simulink model "sm_car"  (R2025a)
settings: Solver=ode23t  StartTime=0.0  StopTime=400  MaxStep=0.4  RelTol=1e-3  AbsTol=1e-3  EnableMultiTasking=on
PreLoadFcn:
  | % Due to usability issue in Repeating Sequence block
  | warning('off','Simulink:Masking:Invalid');
  | 
  | % Eliminate unnecessary warnings in inactive variants
  | % Warnings generated only if you click through inactive variant
  | warning('off','MATLAB:nonExistentField');
  | warning('off','Simulink:Parameters:BlkParamUndefined');
PostLoadFcn:
  | set_param([bdroot '/Vehicle'],'popup_trailer','Off')
  | warning('off','sm:sli:setup:compile:LocalSolverNotSupported')
  | %sm_car_config_maneuver(bdroot,'WOT Braking');
  | sm_car_config_vehicle(bdroot,'false');
  | sm_car_config_logging(bdroot);
InitFcn:
  | sm_car_config_camera;
  | Vehicle = sm_car_vehcfg_checkConfig(Vehicle);
  | sm_car_check_tire_model(bdroot);
StartFcn:
  | tic;
StopFcn:
  | Elapsed_Sim_Time = toc;
  | % disp(['Elapsed Sim Time = ' num2str(Elapsed_Sim_Time)]);
undefined symbols (not defined in the file): Axle1D, AxleIn, Camera, Control, Driver, Free, Init, Maneuver, Pedal, RaceFix, RaceSpin, Scene, ShaftL1, ShaftL2, ShaftR1, ShaftR2, Soft, Stiff, Visual, X, xy_data_car_side, Y, Z
libraries: sm_lib x1546, nesl_utility x528, fl_lib x480, SimscapeFluids_lib x61, sdl_lib x49, simulink x29, ee_lib x7, simulink_extras x6, Linkage_Systems x4, Tire_1x2x x4, AntiRollBar_Systems x2, Linkage_Decoupled x2
(part 55 of 79)

== system sm_car/Vehicle/Vehicle/Chassis/SuspA1/Linkage Decoupled/Steer/Wheel Driven Rack 1UJoint/Steer Mount ==
  note: Two additional degrees of freedom have been added
      | to ensure steering column assembles within tolerances.
  Cylindrical Joint : sm_lib/Joints/Cylindrical Joint  JointMode=Normal  CompositeWrenchDir=FollowerOnBase  CompositeWrenchFrame=BaseFrame  SenseConstraintForce=off  SenseConstraintTorque=off  SenseTotalForce=off  SenseTotalTorque=off  RzPositionTargetSpecify=off  RzPositionTargetPriority=High  RzPositionTargetValue=0  RzPositionTargetValueUnits=deg  RzVelocityTargetSpecify=off  RzVelocityTargetPriority=High  RzVelocityTargetValue=0  RzVelocityTargetValueUnits=deg/s  RzEquilibriumPosition=0  RzEquilibriumPositionUnits=deg  RzSpringStiffness=0  RzSpringStiffnessUnits=N*m/deg  RzDampingCoefficient=0  RzDampingCoefficientUnits=N*m/(deg/s)  RzLowerLimitSpecify=off  RzLowerLimitBound=-90  RzLowerLimitBoundUnits=deg  RzLowerLimitStiffness=1e4  RzLowerLimitStiffnessUnits=N*m/deg  RzLowerLimitDamping=10  RzLowerLimitDampingUnits=N*m/(deg/s)  RzLowerLimitTransitionRegionWidth=0.1  RzLowerLimitTransitionRegionWidthUnits=deg  RzUpperLimitSpecify=off  RzUpperLimitBound=90  RzUpperLimitBoundUnits=deg  RzUpperLimitStiffness=1e4  RzUpperLimitStiffnessUnits=N*m/deg  RzUpperLimitDamping=10  RzUpperLimitDampingUnits=N*m/(deg/s)  RzUpperLimitTransitionRegionWidth=0.1  RzUpperLimitTransitionRegionWidthUnits=deg  RzTorqueActuationMode=ComputedTorque  RzMotionActuationMode=InputMotion  RzSensePosition=on  RzSenseVelocity=off  RzSenseAcceleration=off  RzSenseTorqueForce=off  RzSenseLowerLimitTorqueForce=off  RzSenseUpperLimitTorqueForce=off  PzPositionTargetSpecify=off  PzPositionTargetPriority=High  PzPositionTargetValue=0  PzPositionTargetValueUnits=m  PzVelocityTargetSpecify=off  PzVelocityTargetPriority=High  PzVelocityTargetValue=0  PzVelocityTargetValueUnits=m/s  PzEquilibriumPosition=0  PzEquilibriumPositionUnits=m  PzSpringStiffness=0  PzSpringStiffnessUnits=N/m  PzDampingCoefficient=0  PzDampingCoefficientUnits=N/(m/s)  PzLowerLimitSpecify=off  PzLowerLimitBound=-1  PzLowerLimitBoundUnits=m  PzLowerLimitStiffness=1e6  PzLowerLimitStiffnessUnits=N/m  PzLowerLimitDamping=1e3  PzLowerLimitDampingUnits=N/(m/s)  PzLowerLimitTransitionRegionWidth=1e-4  PzLowerLimitTransitionRegionWidthUnits=m  PzUpperLimitSpecify=off  PzUpperLimitBound=1  PzUpperLimitBoundUnits=m  PzUpperLimitStiffness=1e6  PzUpperLimitStiffnessUnits=N/m  PzUpperLimitDamping=1e3  PzUpperLimitDampingUnits=N/(m/s)  PzUpperLimitTransitionRegionWidth=1e-4  PzUpperLimitTransitionRegionWidthUnits=m  PzTorqueActuationMode=NoTorque  PzMotionActuationMode=ComputedMotion  PzSensePosition=off  PzSenseVelocity=off  PzSenseAcceleration=off  PzSenseTorqueForce=off  PzSenseLowerLimitTorqueForce=off  PzSenseUpperLimitTorqueForce=off
  Revolute Joint : sm_lib/Joints/Revolute Joint  JointMode=Normal  CompositeWrenchDir=FollowerOnBase  CompositeWrenchFrame=BaseFrame  SenseConstraintForce=off  SenseConstraintTorque=off  SenseTotalForce=off  SenseTotalTorque=off  PositionTargetSpecify=off  PositionTargetPriority=High  PositionTargetValue=0  PositionTargetValueUnits=deg  VelocityTargetSpecify=off  VelocityTargetPriority=High  VelocityTargetValue=0  VelocityTargetValueUnits=deg/s  EquilibriumPosition=0  EquilibriumPositionUnits=deg  SpringStiffness=0  SpringStiffnessUnits=N*m/deg  DampingCoefficient=0  DampingCoefficientUnits=N*m/(deg/s)  LowerLimitSpecify=off  LowerLimitBound=-90  LowerLimitBoundUnits=deg  LowerLimitStiffness=1e4  LowerLimitStiffnessUnits=N*m/deg  LowerLimitDamping=10  LowerLimitDampingUnits=N*m/(deg/s)  LowerLimitTransitionRegionWidth=0.1  LowerLimitTransitionRegionWidthUnits=deg  UpperLimitSpecify=off  UpperLimitBound=90  UpperLimitBoundUnits=deg  UpperLimitStiffness=1e4  UpperLimitStiffnessUnits=N*m/deg  UpperLimitDamping=10  UpperLimitDampingUnits=N*m/(deg/s)  UpperLimitTransitionRegionWidth=0.1  UpperLimitTransitionRegionWidthUnits=deg  TorqueActuationMode=NoTorque  MotionActuationMode=ComputedMotion  SensePosition=off  SenseVelocity=off  SenseAcceleration=off  SenseTorqueForce=off  SenseLowerLimitTorqueForce=off  SenseUpperLimitTorqueForce=off
  Transform DOF wy B : sm_lib/Frames and Transforms/Rigid Transform  RotationMethod=StandardAxis  FollAlignAxisA=+X  BaseAlignAxisA=+Y  FollAlignAxisB=+Y  BaseAlignAxisB=+Z  RotationStandardAxis=+X  RotationAngle=-90  RotationAngleUnits=deg  RotationArbitraryAxis=[0 0 1]  RotationSequenceAxes=FollowerAxes  RotationSequence=XYX  RotationSequenceAngles=[0 0 0]  RotationSequenceAnglesUnits=deg  RotationMatrix=[1 0 0; 0 1 0; 0 0 1]  Quaternion=[1 0 0 0]  TranslationMethod=None  TranslationCartesianOffset=[0 0 0]  TranslationCartesianOffsetUnits=m  TranslationStandardAxis=+Z  TranslationStandardOffset=0  TranslationStandardOffsetUnits=m  TranslationROffset=0  TranslationROffsetUnits=m  TranslationThetaOffset=0  TranslationThetaOffsetUnits=deg  TranslationZOffset=0  TranslationZOffsetUnits=m
  Transform DOF wy F : sm_lib/Frames and Transforms/Rigid Transform  RotationMethod=StandardAxis  FollAlignAxisA=+X  BaseAlignAxisA=+Y  FollAlignAxisB=+Y  BaseAlignAxisB=+Z  RotationStandardAxis=+X  RotationAngle=-90  RotationAngleUnits=deg  RotationArbitraryAxis=[0 0 1]  RotationSequenceAxes=FollowerAxes  RotationSequence=XYX  RotationSequenceAngles=[0 0 0]  RotationSequenceAnglesUnits=deg  RotationMatrix=[1 0 0; 0 1 0; 0 0 1]  Quaternion=[1 0 0 0]  TranslationMethod=None  TranslationCartesianOffset=[0 0 0]  TranslationCartesianOffsetUnits=m  TranslationStandardAxis=+Z  TranslationStandardOffset=0  TranslationStandardOffsetUnits=m  TranslationROffset=0  TranslationROffsetUnits=m  TranslationThetaOffset=0  TranslationThetaOffsetUnits=deg  TranslationZOffset=0  TranslationZOffsetUnits=m
  F : PMIOPort  Side=Right
  B : PMIOPort  Port=2  Side=Left
  a : PMIOPort  Port=3  Side=Right
  q : PMIOPort  Port=4  Side=Left
  connections:
  a/RConn1 -- Cylindrical Joint/RConn2
  q/RConn1 -- Cylindrical Joint/LConn2
  Transform DOF wy B/LConn1 -- B/RConn1
  Cylindrical Joint/RConn1 -- F/RConn1
  Cylindrical Joint/LConn1 -- Transform DOF wy F/LConn1
  Revolute Joint/LConn1 -- Transform DOF wy B/RConn1
  Transform DOF wy F/RConn1 -- Revolute Joint/RConn1

== system sm_car/Vehicle/Vehicle/Chassis/SuspA1/Linkage Decoupled/Steer/Wheel Driven Rack 1UJoint/Wheel ==
  FSAE : Subsystem  VariantControl=FSAE
  Sedan : Subsystem  VariantControl=Sedan  mask{clr_wheel=Visual.SteeringWheel.clr, opc_wheel=1}
      mask prompts: clr_wheel "Color [RGB]"; opc_wheel "Opacity (0-1)"
  SteerAxis : PMIOPort  Side=Left
  HandR : PMIOPort  Port=2  Side=Right
  HandL : PMIOPort  Port=3  Side=Right

== system sm_car/Vehicle/Vehicle/Chassis/SuspA2/Linkage/Steer/None/Body Sensor ==
  note: Calculation not yet implemented
  Constant : Constant  Value=0
  Constant1 : Constant  Value=0
  PS-Simulink Converter1 : nesl_utility/PS-Simulink Converter  PhysicalDomain=network_engine_domain  SubClassName=ps_output  LeftPortType=input  RightPortType=output  PseudoPeriodic=off  Frequencies=[]  VectorFormat=1-D array  Unit=m  AffineConversion=off
  PS-Simulink Converter11 : nesl_utility/PS-Simulink Converter  PhysicalDomain=network_engine_domain  SubClassName=ps_output  LeftPortType=input  RightPortType=output  PseudoPeriodic=off  Frequencies=[]  VectorFormat=1-D array  Unit=1  AffineConversion=off
  PS-Simulink Converter2 : nesl_utility/PS-Simulink Converter  PhysicalDomain=network_engine_domain  SubClassName=ps_output  LeftPortType=input  RightPortType=output  PseudoPeriodic=off  Frequencies=[]  VectorFormat=1-D array  Unit=m  AffineConversion=off
  PS-Simulink Converter3 : nesl_utility/PS-Simulink Converter  PhysicalDomain=network_engine_domain  SubClassName=ps_output  LeftPortType=input  RightPortType=output  PseudoPeriodic=off  Frequencies=[]  VectorFormat=1-D array  Unit=m  AffineConversion=off
  PS-Simulink Converter4 : nesl_utility/PS-Simulink Converter  PhysicalDomain=network_engine_domain  SubClassName=ps_output  LeftPortType=input  RightPortType=output  PseudoPeriodic=off  Frequencies=[]  VectorFormat=1-D array  Unit=m/s  AffineConversion=off
  PS-Simulink Converter5 : nesl_utility/PS-Simulink Converter  PhysicalDomain=network_engine_domain  SubClassName=ps_output  LeftPortType=input  RightPortType=output  PseudoPeriodic=off  Frequencies=[]  VectorFormat=1-D array  Unit=m/s  AffineConversion=off
  PS-Simulink Converter6 : nesl_utility/PS-Simulink Converter  PhysicalDomain=network_engine_domain  SubClassName=ps_output  LeftPortType=input  RightPortType=output  PseudoPeriodic=off  Frequencies=[]  VectorFormat=1-D array  Unit=m/s  AffineConversion=off
  PS-Simulink Converter7 : nesl_utility/PS-Simulink Converter  PhysicalDomain=network_engine_domain  SubClassName=ps_output  LeftPortType=input  RightPortType=output  PseudoPeriodic=off  Frequencies=[]  VectorFormat=1-D array  Unit=m/s^2  AffineConversion=off
  PS-Simulink Converter8 : nesl_utility/PS-Simulink Converter  PhysicalDomain=network_engine_domain  SubClassName=ps_output  LeftPortType=input  RightPortType=output  PseudoPeriodic=off  Frequencies=[]  VectorFormat=1-D array  Unit=m/s^2  AffineConversion=off
  PS-Simulink Converter9 : nesl_utility/PS-Simulink Converter  PhysicalDomain=network_engine_domain  SubClassName=ps_output  LeftPortType=input  RightPortType=output  PseudoPeriodic=off  Frequencies=[]  VectorFormat=1-D array  Unit=m/s^2  AffineConversion=off
  Roll Pitch : Subsystem
  Signal Specification : SignalSpecification  Unit=rad
  Signal Specification1 : SignalSpecification  Unit=rad
  Signal Specification2 : SignalSpecification  Unit=rad
  Signal Specification3 : SignalSpecification  Unit=rad/s
  Signal Specification4 : SignalSpecification  Unit=rad/s
  Signal Specification5 : SignalSpecification  Unit=rad/s
  Transform Sensor Offset : sm_lib/Frames and Transforms/Rigid Transform  RotationMethod=None  FollAlignAxisA=+X  BaseAlignAxisA=+Y  FollAlignAxisB=+Y  BaseAlignAxisB=+Z  RotationStandardAxis=+Z  RotationAngle=0.0  RotationAngleUnits=deg  RotationArbitraryAxis=[0 0 1]  RotationSequenceAxes=FollowerAxes  RotationSequence=XYX  RotationSequenceAngles=[0 0 0]  RotationSequenceAnglesUnits=deg  RotationMatrix=[1 0 0; 0 1 0; 0 0 1]  Quaternion=[1 0 0 0]  TranslationMethod=Cartesian  TranslationCartesianOffset=offset_body_sensor  TranslationCartesianOffsetUnits=m  TranslationStandardAxis=+Z  TranslationStandardOffset=0  TranslationStandardOffsetUnits=m  TranslationROffset=0  TranslationROffsetUnits=m  TranslationThetaOffset=0  TranslationThetaOffsetUnits=deg  TranslationZOffset=0  TranslationZOffsetUnits=m
  Transform Sensor Body : sm_lib/Frames and Transforms/Transform Sensor  MeasurementFrame=NonRotatingFollower  RotationSequence=XYX  SenseAngle=off  SenseAxis=off  SenseQ=off  SenseR=on  SenseRotationSequence=off  SenseOmegaX=off  SenseOmegaY=off  SenseOmegaZ=off  SenseOmega=off  SenseQDot=off  SenseRDot=off  SenseRotationSequenceDot=off  SenseAlphaX=off  SenseAlphaY=off  SenseAlphaZ=off  SenseAlpha=off  SenseQDDot=off  SenseRDDot=off  SenseX=on  SenseY=on  SenseZ=on  SenseXYZ=off  SenseRad=off  SenseAzim=off  SenseDist=off  SenseInc=off  SenseXDot=on  SenseYDot=on  SenseZDot=on  SenseXYZDot=off  SenseRadDot=off  SenseAzimDot=off  SenseDistDot=off  SenseIncDot=off  SenseXDDot=on  SenseYDDot=on  SenseZDDot=on  SenseXYZDDot=off  SenseRadDDot=off  SenseAzimDDot=off  SenseDistDDot=off  SenseIncDDot=off
  World Frame : sm_lib/Frames and Transforms/World Frame
  B : PMIOPort  Side=Left
  Bus Element Out : Outport  VectorParamsAs1DForOutWhenUnconnected=off  PortName=Body  Element=x
  Bus Element Out1 : Outport  VectorParamsAs1DForOutWhenUnconnected=off  PortName=Body  Element=y
  Bus Element Out2 : Outport  VectorParamsAs1DForOutWhenUnconnected=off  PortName=Body  Element=z
  Bus Element Out3 : Outport  VectorParamsAs1DForOutWhenUnconnected=off  PortName=Body  Element=vx
  Bus Element Out4 : Outport  VectorParamsAs1DForOutWhenUnconnected=off  PortName=Body  Element=vy
  Bus Element Out5 : Outport  VectorParamsAs1DForOutWhenUnconnected=off  PortName=Body  Element=vz
  Bus Element Out6 : Outport  VectorParamsAs1DForOutWhenUnconnected=off  PortName=Body  Element=gx
  Bus Element Out7 : Outport  VectorParamsAs1DForOutWhenUnconnected=off  PortName=Body  Element=gy
  Bus Element Out8 : Outport  VectorParamsAs1DForOutWhenUnconnected=off  PortName=Body  Element=gz
  Bus Element Out9 : Outport  VectorParamsAs1DForOutWhenUnconnected=off  PortName=Body  Element=nRoll
  Bus Element Out10 : Outport  VectorParamsAs1DForOutWhenUnconnected=off  PortName=Body  Element=nPitch
  Bus Element Out11 : Outport  VectorParamsAs1DForOutWhenUnconnected=off  PortName=Body  Element=nYaw
  Bus Element Out12 : Outport  VectorParamsAs1DForOutWhenUnconnected=off  PortName=Body  Element=aRoll
  Bus Element Out13 : Outport  VectorParamsAs1DForOutWhenUnconnected=off  PortName=Body  Element=aPitch
  Bus Element Out14 : Outport  VectorParamsAs1DForOutWhenUnconnected=off  PortName=Body  Element=aYaw
  wires:
  PS-Simulink Converter9/1 -> Bus Element Out8/1
  PS-Simulink Converter11/1 -> Roll Pitch/1(R)
  PS-Simulink Converter6/1 -> Bus Element Out5/1
  PS-Simulink Converter7/1 -> Bus Element Out6/1
  PS-Simulink Converter2/1 -> Bus Element Out1/1
  PS-Simulink Converter8/1 -> Bus Element Out7/1
  PS-Simulink Converter5/1 -> Bus Element Out4/1
  PS-Simulink Converter3/1 -> Bus Element Out2/1
  PS-Simulink Converter1/1 -> Bus Element Out/1
  PS-Simulink Converter4/1 -> Bus Element Out3/1
  Signal Specification/1 -> Bus Element Out12/1
  Signal Specification1/1 -> Bus Element Out13/1
  Signal Specification2/1 -> Bus Element Out14/1
  Signal Specification3/1 -> Bus Element Out9/1
  Signal Specification4/1 -> Bus Element Out10/1
  Signal Specification5/1 -> Bus Element Out11/1
  Constant/1 -> Signal Specification2/1
  Constant1/1 -> Signal Specification5/1
  Roll Pitch/3(nRoll) -> Signal Specification3/1
  Roll Pitch/4(nPitch) -> Signal Specification4/1
  Roll Pitch/2(aPitch) -> Signal Specification1/1
  Roll Pitch/1(aRoll) -> Signal Specification/1
  connections:
  Transform Sensor Body/RConn5 -- PS-Simulink Converter3/LConn1
  Transform Sensor Body/RConn4 -- PS-Simulink Converter2/LConn1
  Transform Sensor Body/RConn11 -- PS-Simulink Converter9/LConn1
  Transform Sensor Body/RConn2 -- PS-Simulink Converter11/LConn1
  Transform Sensor Body/RConn7 -- PS-Simulink Converter5/LConn1
  Transform Sensor Body/RConn3 -- PS-Simulink Converter1/LConn1
  Transform Sensor Body/LConn1 -- World Frame/RConn1
  Transform Sensor Offset/LConn1 -- B/RConn1
  Transform Sensor Body/RConn10 -- PS-Simulink Converter8/LConn1
  Transform Sensor Body/RConn9 -- PS-Simulink Converter7/LConn1
  Transform Sensor Body/RConn8 -- PS-Simulink Converter6/LConn1
  Transform Sensor Body/RConn6 -- PS-Simulink Converter4/LConn1
  Transform Sensor Body/RConn1 -- Transform Sensor Offset/RConn1

== system sm_car/Vehicle/Vehicle/Powertrain/Power/Electric L1 R1 L2 R2/Thermal/Liquid Loop1/Pump Control ==
  T : Inport
  Memory : Memory
  Pump Time Constant : TransferFcn  Denominator=[0.1 1]
  Relay : Relay  OnSwitchValue=313  OffSwitchValue=293  ZeroCross=off
  M : Outport  VectorParamsAs1DForOutWhenUnconnected=off
  wires:
  Pump Time Constant/1 -> M/1
  Memory/1 -> Relay/1
  T/1 -> Memory/1
  Relay/1 -> Pump Time Constant/1  "Pump_flw"

== system sm_car/Vehicle/Vehicle/Powertrain/Power/Electric L1 R1 L2 R2/Thermal/Liquid Loop1/Sensing TBattery ==
  PS-Simulink Converter4 : nesl_utility/PS-Simulink Converter  PhysicalDomain=network_engine_domain  SubClassName=ps_output  LeftPortType=input  RightPortType=output  PseudoPeriodic=off  Frequencies=[]  VectorFormat=1-D array  Unit=K  AffineConversion=on
  Temperature Sensor : fl_lib/Thermal/Thermal Sensors/Temperature Sensor  temperature_measure=foundation.enum.MeasurementReference.difference
  Thermal Reference : fl_lib/Thermal/Thermal Elements/Thermal Reference
  A : PMIOPort  Side=Left
  T : Outport  VectorParamsAs1DForOutWhenUnconnected=off
  wires:
  PS-Simulink Converter4/1 -> T/1  "Temperature"
  connections:
  Temperature Sensor/LConn1 -- A/RConn1
  Thermal Reference/LConn1 -- Temperature Sensor/RConn1
  Temperature Sensor/RConn2 -- PS-Simulink Converter4/LConn1

== system sm_car/Vehicle/Vehicle/Powertrain/Power/Electric L1 R1 L2 R2/Thermal/Liquid Loop1/Sensing TConverter ==
  PS-Simulink Converter4 : nesl_utility/PS-Simulink Converter  PhysicalDomain=network_engine_domain  SubClassName=ps_output  LeftPortType=input  RightPortType=output  PseudoPeriodic=off  Frequencies=[]  VectorFormat=1-D array  Unit=K  AffineConversion=on
  Temperature Sensor : fl_lib/Thermal/Thermal Sensors/Temperature Sensor  temperature_measure=foundation.enum.MeasurementReference.difference
  Thermal Reference : fl_lib/Thermal/Thermal Elements/Thermal Reference
  A : PMIOPort  Side=Left
  T : Outport  VectorParamsAs1DForOutWhenUnconnected=off
  wires:
  PS-Simulink Converter4/1 -> T/1  "Temperature"
  connections:
  Temperature Sensor/RConn2 -- PS-Simulink Converter4/LConn1
  Thermal Reference/LConn1 -- Temperature Sensor/RConn1
  Temperature Sensor/LConn1 -- A/RConn1

== system sm_car/Vehicle/Vehicle/Powertrain/Power/Electric L1 R1 L2 R2/Thermal/Liquid Loop1/Sensing TMotorR1 ==
  PS-Simulink Converter4 : nesl_utility/PS-Simulink Converter  PhysicalDomain=network_engine_domain  SubClassName=ps_output  LeftPortType=input  RightPortType=output  PseudoPeriodic=off  Frequencies=[]  VectorFormat=1-D array  Unit=K  AffineConversion=on
  Temperature Sensor : fl_lib/Thermal/Thermal Sensors/Temperature Sensor  temperature_measure=foundation.enum.MeasurementReference.difference
  Thermal Reference : fl_lib/Thermal/Thermal Elements/Thermal Reference
  A : PMIOPort  Side=Left
  T : Outport  VectorParamsAs1DForOutWhenUnconnected=off
  wires:
  PS-Simulink Converter4/1 -> T/1  "Temperature"
  connections:
  Temperature Sensor/RConn2 -- PS-Simulink Converter4/LConn1
  Thermal Reference/LConn1 -- Temperature Sensor/RConn1
  Temperature Sensor/LConn1 -- A/RConn1

== system sm_car/Vehicle/Vehicle/Powertrain/Power/Electric L1 R1 L2 R2/Thermal/Liquid Loop1/Sensing TMotorRL ==
  PS-Simulink Converter4 : nesl_utility/PS-Simulink Converter  PhysicalDomain=network_engine_domain  SubClassName=ps_output  LeftPortType=input  RightPortType=output  PseudoPeriodic=off  Frequencies=[]  VectorFormat=1-D array  Unit=K  AffineConversion=on
  Temperature Sensor : fl_lib/Thermal/Thermal Sensors/Temperature Sensor  temperature_measure=foundation.enum.MeasurementReference.difference
  Thermal Reference : fl_lib/Thermal/Thermal Elements/Thermal Reference
  A : PMIOPort  Side=Left
  T : Outport  VectorParamsAs1DForOutWhenUnconnected=off
  wires:
  PS-Simulink Converter4/1 -> T/1  "Temperature"
  connections:
  Temperature Sensor/LConn1 -- A/RConn1
  Thermal Reference/LConn1 -- Temperature Sensor/RConn1
  Temperature Sensor/RConn2 -- PS-Simulink Converter4/LConn1

== system sm_car/Vehicle/Vehicle/Powertrain/Power/Electric L1 R1 L2 R2/Thermal/Liquid Loop1/Sensing TMotorRL1 ==
  PS-Simulink Converter4 : nesl_utility/PS-Simulink Converter  PhysicalDomain=network_engine_domain  SubClassName=ps_output  LeftPortType=input  RightPortType=output  PseudoPeriodic=off  Frequencies=[]  VectorFormat=1-D array  Unit=K  AffineConversion=on
  Temperature Sensor : fl_lib/Thermal/Thermal Sensors/Temperature Sensor  temperature_measure=foundation.enum.MeasurementReference.difference
  Thermal Reference : fl_lib/Thermal/Thermal Elements/Thermal Reference
  A : PMIOPort  Side=Left
  T : Outport  VectorParamsAs1DForOutWhenUnconnected=off
  wires:
  PS-Simulink Converter4/1 -> T/1  "Temperature"
  connections:
  Temperature Sensor/RConn2 -- PS-Simulink Converter4/LConn1
  Thermal Reference/LConn1 -- Temperature Sensor/RConn1
  Temperature Sensor/LConn1 -- A/RConn1

== system sm_car/Vehicle/Vehicle/Powertrain/Power/Electric L1 R1 L2 R2/Thermal/Liquid Loop1/Sensing TMotorRR ==
  PS-Simulink Converter4 : nesl_utility/PS-Simulink Converter  PhysicalDomain=network_engine_domain  SubClassName=ps_output  LeftPortType=input  RightPortType=output  PseudoPeriodic=off  Frequencies=[]  VectorFormat=1-D array  Unit=K  AffineConversion=on
  Temperature Sensor : fl_lib/Thermal/Thermal Sensors/Temperature Sensor  temperature_measure=foundation.enum.MeasurementReference.difference
  Thermal Reference : fl_lib/Thermal/Thermal Elements/Thermal Reference
  A : PMIOPort  Side=Left
  T : Outport  VectorParamsAs1DForOutWhenUnconnected=off
  wires:
  PS-Simulink Converter4/1 -> T/1  "Temperature"
  connections:
  Temperature Sensor/LConn1 -- A/RConn1
  Thermal Reference/LConn1 -- Temperature Sensor/RConn1
  Temperature Sensor/RConn2 -- PS-Simulink Converter4/LConn1

== system sm_car/Vehicle/Vehicle/Powertrain/Power/Electric L1 R1 L2 R2/Thermal/Liquid Loop1/Tank ==
  Absolute Reference (TL) : fl_lib/Thermal Liquid/Elements/Absolute Reference (TL)
  Cap (G) : fl_lib/Gas/Elements/Cap (G)  p_specify=off  p_priority=None  p=0.101325 MPa  p_nominal_specify=off  p_nominal_value=1  p_nominal_unit=MPa  T_specify=off  T_priority=None  T=293.15 K  T_nominal_specify=off  T_nominal_value=1  T_nominal_unit=K
  Convective Heat Transfer : fl_lib/Thermal/Thermal Elements/Convective Heat Transfer  thermal_type=foundation.enum.constant_variable.constant  area=1 m^2  heat_tr_coeff=20 W/(m^2 * K)  min_heat_tr_coeff=1e-3 W/(K*m^2)  T_specify=off  T_priority=None  T=0 K  T_nominal_specify=off  T_nominal_value=1  T_nominal_unit=K  Q_specify=off  Q_priority=None  Q=0 W  Q_nominal_specify=off  Q_nominal_value=1  Q_nominal_unit=W
  Convective Heat Transfer1 : fl_lib/Thermal/Thermal Elements/Convective Heat Transfer  thermal_type=foundation.enum.constant_variable.constant  area=1 m^2  heat_tr_coeff=200 W/(m^2 * K)  min_heat_tr_coeff=1e-3 W/(K*m^2)  T_specify=off  T_priority=None  T=0 K  T_nominal_specify=off  T_nominal_value=1  T_nominal_unit=K  Q_specify=off  Q_priority=None  Q=0 W  Q_nominal_specify=off  Q_nominal_value=1  Q_nominal_unit=W
  PS Terminator : fl_lib/Physical Signals/Sinks/PS Terminator
  PS Terminator1 : fl_lib/Physical Signals/Sinks/PS Terminator
  PS Terminator2 : fl_lib/Physical Signals/Sinks/PS Terminator
  Reservoir (G) : fl_lib/Gas/Elements/Reservoir (G)  pressure_spec=1  reservoir_pressure=0.101325 MPa  reservoir_temperature=25 degC  area_A=0.001 m^2
  Sensor P T : fl_lib/Thermal Liquid/Sensors/Pressure & Temperature Sensor (TL)  reference=foundation.enum.MeasurementReference.difference  pressure=true  pressure_spec=foundation.enum.PressureMeasementSpec.Absolute  temperature=true
      settings: InternalSimscapePortConfiguration="{\"Bottom\":[{\"id\":\"T\",\"label\":\"T\",\"type\":\"output\"}],\"Left\":[{\"id\":\"A\",\"label\":\"A\",\"type\":\"foundation.thermal_liquid.thermal_liquid\"}],\"Right\":[{\"id\":\"B\",\"label\":\"B\",\"type\":\"foundation.thermal_liquid.thermal_liquid\"},{\"id\":\"P\",\"label\":\"P\",\"type\":\"output\"}],\"Top\":[]}"
  Tank : SimscapeFluids_lib/Thermal Liquid/Tanks & Accumulators/Tank (G-TL)  num_inlet=2  volume_total=0.01 m^3  volume_spec=1  tank_area=0.005 m^2  level_TLU=[0, 3, 5] m  volume_TLU=[0, 4, 6] m^3  inlet_areas_A1B1=[.001, .001] m^2  inlet_height_A2=0.1 m  inlet_area_A2=0.01 m^2  inlet_heights_A2B2=[.01, 0.01] m  inlet_areas_A2B2=[0.01^2/4*pi, 0.01^2/4*pi] m^2  inlet_heights_A2B2C2=[.1, .1, .1] m  inlet_areas_A2B2C2=[.01, .01, .01] m^2  inlet_heights_A2B2C2D2=0.1 * ones(1, 4) m  inlet_areas_A2B2C2D2=0.01 * ones(1, 4) m^2  inlet_heights_A2B2C2D2E2=0.1 * ones(1, 5) m  inlet_areas_A2B2C2D2E2=0.01 * ones(1, 5) m^2  inlet_heights_A2B2C2D2E2F2=0.1 * ones(1, 6) m  inlet_areas_A2B2C2D2E2F2=0.01 * ones(1, 6) m^2  capacity_check=0  max_liquid_capacity=0.01 m^3  g=9.81 m/s^2  level_specify=on  level_priority=High  level=0.1 m  level_nominal_specify=off  level_nominal_value=1  level_nominal_unit=m  volume_liquid_specify=off  volume_liquid_priority=None  volume_liquid=5 m^3  volume_liquid_nominal_specify=off  volume_liquid_nominal_value=1  volume_liquid_nominal_unit=m^3  mass_liquid_specify=off  mass_liquid_priority=None  mass_liquid=5e+3 kg  mass_liquid_nominal_specify=off  mass_liquid_nominal_value=1  mass_liquid_nominal_unit=kg  T_liquid_specify=on  T_liquid_priority=High  T_liquid=278 K  T_liquid_nominal_specify=off  T_liquid_nominal_value=1  T_liquid_nominal_unit=K  p_gas_specify=off  p_gas_priority=High  p_gas=0.101325 MPa  p_gas_nominal_specify=off  p_gas_nominal_value=1  p_gas_nominal_unit=MPa  T_gas_specify=on  T_gas_priority=High  T_gas=278 K  T_gas_nominal_specify=off  T_gas_nominal_value=1  T_gas_nominal_unit=K  rho_gas_specify=off  rho_gas_priority=None  rho_gas=1.2 kg/m^3  rho_gas_nominal_specify=off  rho_gas_nominal_value=1  rho_gas_nominal_unit=kg/m^3
      settings: InternalSimscapePortConfiguration="{\"Bottom\":[],\"Left\":[{\"id\":\"A1\",\"label\":\"A1\",\"type\":\"foundation.gas.gas\"},{\"id\":\"B1\",\"label\":\"B1\",\"type\":\"foundation.gas.gas\"},{\"id\":\"A2\",\"label\":\"A2\",\"type\":\"foundation.thermal_liquid.thermal_liquid\"},{\"id\":\"B2\",\"label\":\"B2\",\"type\":\"foundation.thermal_liquid.thermal_liquid\"}],\"Right\":[{\"id\":\"H1\",\"label\":\"H1\",\"type\":\"foundation.thermal.thermal\"},{\"id\":\"H2\",\"label\":\"H2\",\"type\":\"foundation.thermal.thermal\"}],\"Top\":[{\"id\":\"V_out\",\"label\":\"V\",\"type\":\"output\"},{\"id\":\"L_out\",\"label\":\"L\",\"type\":\"output\"}]}"
  B : PMIOPort  Side=Left
  HGas : PMIOPort  Port=2  Side=Left
  A : PMIOPort  Port=3  Side=Right
  T : PMIOPort  Port=4  Side=Right
  HLiq : PMIOPort  Port=5  Side=Left
  connections:
  HLiq/RConn1 -- Convective Heat Transfer1/RConn1
  Convective Heat Transfer/LConn1 -- Tank/RConn1
  HGas/RConn1 -- Convective Heat Transfer/RConn1
  Sensor P T/RConn2 -- PS Terminator2/LConn1
  Cap (G)/LConn1 -- Tank/LConn2
  Tank/LConn3 -- A/RConn1
  Reservoir (G)/LConn1 -- Tank/LConn1
  Absolute Reference (TL)/LConn1 -- Sensor P T/RConn1
  Sensor P T/RConn3 -- T/RConn1
  Tank/LConn4 -- B/RConn1 -- Sensor P T/LConn1
  Convective Heat Transfer1/LConn1 -- Tank/RConn2
  Tank/LConn5 -- PS Terminator/LConn1
  Tank/LConn6 -- PS Terminator1/LConn1

== system sm_car/Vehicle/Vehicle/Powertrain/Power/Electric L1 R1 L2 R2/Thermal/Liquid Loop1/Thermal Circuit Battery ==
  Conductive Heat Transfer : fl_lib/Thermal/Thermal Elements/Conductive Heat Transfer  thermal_type=foundation.enum.ConstantVariableTabulated.Constant  wall_geometry=foundation.enum.ConductionWallGeometry.Planar  area=pi m^2  thickness=0.004 m  d_in=0.05 m  d_out=0.1 m  L=1 m  th_cond_min=10 W/(K*m)  th_cond="237;  %Al W/(m*K)"  th_cond_TLU=[413, 401, 392, 383, 371, 357, 342] W/(K*m)  temp_TLU=[200, 273, 400, 600, 800, 1000, 1200] K  T_specify=off  T_priority=None  T=0 K  T_nominal_specify=off  T_nominal_value=1  T_nominal_unit=K  Q_specify=off  Q_priority=None  Q=0 W  Q_nominal_specify=off  Q_nominal_value=1  Q_nominal_unit=W
  Thermal Mass : fl_lib/Thermal/Thermal Elements/Thermal Mass  mass_type=foundation.enum.constant_variable.constant  mass=2 kg  sp_heat=910 J/kg/K  mass_min=1e-6 kg  num_ports=foundation.enum.numPorts2.one  m_specify=off  m_priority=High  m=1 kg  m_nominal_specify=off  m_nominal_value=1  m_nominal_unit=kg  T_specify=off  T_priority=High  T=300 K  T_nominal_specify=off  T_nominal_value=1  T_nominal_unit=K  Q_specify=off  Q_priority=None  Q=0 W  Q_nominal_specify=off  Q_nominal_value=1  Q_nominal_unit=W
  A : PMIOPort  Side=Left
  B : PMIOPort  Port=2  Side=Right
  connections:
  A/RConn1 -- Conductive Heat Transfer/LConn1
  Conductive Heat Transfer/RConn1 -- B/RConn1 -- Thermal Mass/LConn1

== system sm_car/Vehicle/Vehicle/Powertrain/Power/Electric L1 R1 L2 R2/Thermal/Liquid Loop1/Thermal Circuit Converter ==
  Conductive Heat Transfer : fl_lib/Thermal/Thermal Elements/Conductive Heat Transfer  thermal_type=foundation.enum.ConstantVariableTabulated.Constant  wall_geometry=foundation.enum.ConductionWallGeometry.Planar  area=0.01*pi*1 m^2  thickness=0.004 m  d_in=0.05 m  d_out=0.1 m  L=1 m  th_cond_min=10 W/(K*m)  th_cond="237;  %Al W/(m*K)"  th_cond_TLU=[413, 401, 392, 383, 371, 357, 342] W/(K*m)  temp_TLU=[200, 273, 400, 600, 800, 1000, 1200] K  T_specify=off  T_priority=None  T=0 K  T_nominal_specify=off  T_nominal_value=1  T_nominal_unit=K  Q_specify=off  Q_priority=None  Q=0 W  Q_nominal_specify=off  Q_nominal_value=1  Q_nominal_unit=W
  Thermal Mass : fl_lib/Thermal/Thermal Elements/Thermal Mass  mass_type=foundation.enum.constant_variable.constant  mass=2 kg  sp_heat=910 J/kg/K  mass_min=1e-6 kg  num_ports=foundation.enum.numPorts2.one  m_specify=off  m_priority=High  m=1 kg  m_nominal_specify=off  m_nominal_value=1  m_nominal_unit=kg  T_specify=off  T_priority=High  T=300 K  T_nominal_specify=off  T_nominal_value=1  T_nominal_unit=K  Q_specify=off  Q_priority=None  Q=0 W  Q_nominal_specify=off  Q_nominal_value=1  Q_nominal_unit=W
  A : PMIOPort  Side=Left
  B : PMIOPort  Port=2  Side=Right
  connections:
  A/RConn1 -- Conductive Heat Transfer/LConn1
  B/RConn1 -- Conductive Heat Transfer/RConn1 -- Thermal Mass/LConn1

== system sm_car/Vehicle/Vehicle/Powertrain/Power/Electric L1 R1 L2 R2/Thermal/Liquid Loop1/Thermal Circuit Motor L1 ==
  Case-Ambient Insulated : fl_lib/Thermal/Thermal Elements/Perfect Insulator  T_specify=off  T_priority=None  T=0 K  T_nominal_specify=off  T_nominal_value=1  T_nominal_unit=K
  Iron Stack-Case Conductance : fl_lib/Thermal/Thermal Elements/Conductive Heat Transfer  thermal_type=foundation.enum.ConstantVariableTabulated.Constant  wall_geometry=foundation.enum.ConductionWallGeometry.Planar  area=4350 cm^2  thickness=1 cm  d_in=0.05 m  d_out=0.1 m  L=1 m  th_cond_min=10 W/(K*m)  th_cond=80.2 W/(m*K)  th_cond_TLU=[413, 401, 392, 383, 371, 357, 342] W/(K*m)  temp_TLU=[200, 273, 400, 600, 800, 1000, 1200] K  T_specify=off  T_priority=None  T=0 K  T_nominal_specify=off  T_nominal_value=1  T_nominal_unit=K  Q_specify=off  Q_priority=None  Q=0 W  Q_nominal_specify=off  Q_nominal_value=1  Q_nominal_unit=W
  Motor Case Thermal Mass : fl_lib/Thermal/Thermal Elements/Thermal Mass  mass_type=foundation.enum.constant_variable.constant  mass=5 kg  sp_heat=903 J/kg/K  mass_min=1e-6 kg  num_ports=foundation.enum.numPorts2.one  m_specify=off  m_priority=High  m=1 kg  m_nominal_specify=off  m_nominal_value=1  m_nominal_unit=kg  T_specify=off  T_priority=High  T=300 K  T_nominal_specify=off  T_nominal_value=1  T_nominal_unit=K  Q_specify=off  Q_priority=None  Q=0 W  Q_nominal_specify=off  Q_nominal_value=1  Q_nominal_unit=W
  Stator Iron Thermal Mass : fl_lib/Thermal/Thermal Elements/Thermal Mass  mass_type=foundation.enum.constant_variable.constant  mass=5 kg  sp_heat=447 J/kg/K  mass_min=1e-6 kg  num_ports=foundation.enum.numPorts2.one  m_specify=off  m_priority=High  m=1 kg  m_nominal_specify=off  m_nominal_value=1  m_nominal_unit=kg  T_specify=off  T_priority=High  T=300 K  T_nominal_specify=off  T_nominal_value=1  T_nominal_unit=K  Q_specify=off  Q_priority=None  Q=0 W  Q_nominal_specify=off  Q_nominal_value=1  Q_nominal_unit=W
  Winding Conductance : fl_lib/Thermal/Thermal Elements/Conductive Heat Transfer  thermal_type=foundation.enum.ConstantVariableTabulated.Constant  wall_geometry=foundation.enum.ConductionWallGeometry.Planar  area=250.2 cm^2  thickness=1 cm  d_in=0.05 m  d_out=0.1 m  L=1 m  th_cond_min=10 W/(K*m)  th_cond=401 W/(m*K)  th_cond_TLU=[413, 401, 392, 383, 371, 357, 342] W/(K*m)  temp_TLU=[200, 273, 400, 600, 800, 1000, 1200] K  T_specify=off  T_priority=None  T=0 K  T_nominal_specify=off  T_nominal_value=1  T_nominal_unit=K  Q_specify=off  Q_priority=None  Q=0 W  Q_nominal_specify=off  Q_nominal_value=1  Q_nominal_unit=W
  Winding Thermal Mass : fl_lib/Thermal/Thermal Elements/Thermal Mass  mass_type=foundation.enum.constant_variable.constant  mass=5 kg  sp_heat=385 J/kg/K  mass_min=1e-6 kg  num_ports=foundation.enum.numPorts2.one  m_specify=off  m_priority=High  m=1 kg  m_nominal_specify=off  m_nominal_value=1  m_nominal_unit=kg  T_specify=off  T_priority=High  T=300 K  T_nominal_specify=off  T_nominal_value=1  T_nominal_unit=K  Q_specify=off  Q_priority=None  Q=0 W  Q_nominal_specify=off  Q_nominal_value=1  Q_nominal_unit=W
  Winding-Iron Conductance : fl_lib/Thermal/Thermal Elements/Conductive Heat Transfer  thermal_type=foundation.enum.ConstantVariableTabulated.Constant  wall_geometry=foundation.enum.ConductionWallGeometry.Planar  area=250 cm^2  thickness=1 cm  d_in=0.05 m  d_out=0.1 m  L=1 m  th_cond_min=10 W/(K*m)  th_cond=360 W/(m*K)  th_cond_TLU=[413, 401, 392, 383, 371, 357, 342] W/(K*m)  temp_TLU=[200, 273, 400, 600, 800, 1000, 1200] K  T_specify=off  T_priority=None  T=0 K  T_nominal_specify=off  T_nominal_value=1  T_nominal_unit=K  Q_specify=off  Q_priority=None  Q=0 W  Q_nominal_specify=off  Q_nominal_value=1  Q_nominal_unit=W
  A : PMIOPort  Side=Left
  B : PMIOPort  Port=2  Side=Right
  connections:
  Winding Conductance/RConn1 -- A/RConn1
  B/RConn1 -- Winding-Iron Conductance/RConn1 -- Iron Stack-Case Conductance/LConn1 -- Stator Iron Thermal Mass/LConn1
  Case-Ambient Insulated/LConn1 -- Iron Stack-Case Conductance/RConn1 -- Motor Case Thermal Mass/LConn1
  Winding Thermal Mass/LConn1 -- Winding Conductance/LConn1 -- Winding-Iron Conductance/LConn1

== system sm_car/Vehicle/Vehicle/Powertrain/Power/Electric L1 R1 L2 R2/Thermal/Liquid Loop1/Thermal Circuit Motor L2 ==
  Case-Ambient Insulated : fl_lib/Thermal/Thermal Elements/Perfect Insulator  T_specify=off  T_priority=None  T=0 K  T_nominal_specify=off  T_nominal_value=1  T_nominal_unit=K
  Iron Stack-Case Conductance : fl_lib/Thermal/Thermal Elements/Conductive Heat Transfer  thermal_type=foundation.enum.ConstantVariableTabulated.Constant  wall_geometry=foundation.enum.ConductionWallGeometry.Planar  area=4350 cm^2  thickness=1 cm  d_in=0.05 m  d_out=0.1 m  L=1 m  th_cond_min=10 W/(K*m)  th_cond=80.2 W/(m*K)  th_cond_TLU=[413, 401, 392, 383, 371, 357, 342] W/(K*m)  temp_TLU=[200, 273, 400, 600, 800, 1000, 1200] K  T_specify=off  T_priority=None  T=0 K  T_nominal_specify=off  T_nominal_value=1  T_nominal_unit=K  Q_specify=off  Q_priority=None  Q=0 W  Q_nominal_specify=off  Q_nominal_value=1  Q_nominal_unit=W
  Motor Case Thermal Mass : fl_lib/Thermal/Thermal Elements/Thermal Mass  mass_type=foundation.enum.constant_variable.constant  mass=5 kg  sp_heat=903 J/kg/K  mass_min=1e-6 kg  num_ports=foundation.enum.numPorts2.one  m_specify=off  m_priority=High  m=1 kg  m_nominal_specify=off  m_nominal_value=1  m_nominal_unit=kg  T_specify=off  T_priority=High  T=300 K  T_nominal_specify=off  T_nominal_value=1  T_nominal_unit=K  Q_specify=off  Q_priority=None  Q=0 W  Q_nominal_specify=off  Q_nominal_value=1  Q_nominal_unit=W
  Stator Iron Thermal Mass : fl_lib/Thermal/Thermal Elements/Thermal Mass  mass_type=foundation.enum.constant_variable.constant  mass=5 kg  sp_heat=447 J/kg/K  mass_min=1e-6 kg  num_ports=foundation.enum.numPorts2.one  m_specify=off  m_priority=High  m=1 kg  m_nominal_specify=off  m_nominal_value=1  m_nominal_unit=kg  T_specify=off  T_priority=High  T=300 K  T_nominal_specify=off  T_nominal_value=1  T_nominal_unit=K  Q_specify=off  Q_priority=None  Q=0 W  Q_nominal_specify=off  Q_nominal_value=1  Q_nominal_unit=W
  Winding Conductance : fl_lib/Thermal/Thermal Elements/Conductive Heat Transfer  thermal_type=foundation.enum.ConstantVariableTabulated.Constant  wall_geometry=foundation.enum.ConductionWallGeometry.Planar  area=250.2 cm^2  thickness=1 cm  d_in=0.05 m  d_out=0.1 m  L=1 m  th_cond_min=10 W/(K*m)  th_cond=401 W/(m*K)  th_cond_TLU=[413, 401, 392, 383, 371, 357, 342] W/(K*m)  temp_TLU=[200, 273, 400, 600, 800, 1000, 1200] K  T_specify=off  T_priority=None  T=0 K  T_nominal_specify=off  T_nominal_value=1  T_nominal_unit=K  Q_specify=off  Q_priority=None  Q=0 W  Q_nominal_specify=off  Q_nominal_value=1  Q_nominal_unit=W
  Winding Thermal Mass : fl_lib/Thermal/Thermal Elements/Thermal Mass  mass_type=foundation.enum.constant_variable.constant  mass=5 kg  sp_heat=385 J/kg/K  mass_min=1e-6 kg  num_ports=foundation.enum.numPorts2.one  m_specify=off  m_priority=High  m=1 kg  m_nominal_specify=off  m_nominal_value=1  m_nominal_unit=kg  T_specify=off  T_priority=High  T=300 K  T_nominal_specify=off  T_nominal_value=1  T_nominal_unit=K  Q_specify=off  Q_priority=None  Q=0 W  Q_nominal_specify=off  Q_nominal_value=1  Q_nominal_unit=W
  Winding-Iron Conductance : fl_lib/Thermal/Thermal Elements/Conductive Heat Transfer  thermal_type=foundation.enum.ConstantVariableTabulated.Constant  wall_geometry=foundation.enum.ConductionWallGeometry.Planar  area=250 cm^2  thickness=1 cm  d_in=0.05 m  d_out=0.1 m  L=1 m  th_cond_min=10 W/(K*m)  th_cond=360 W/(m*K)  th_cond_TLU=[413, 401, 392, 383, 371, 357, 342] W/(K*m)  temp_TLU=[200, 273, 400, 600, 800, 1000, 1200] K  T_specify=off  T_priority=None  T=0 K  T_nominal_specify=off  T_nominal_value=1  T_nominal_unit=K  Q_specify=off  Q_priority=None  Q=0 W  Q_nominal_specify=off  Q_nominal_value=1  Q_nominal_unit=W
  A : PMIOPort  Side=Left
  B : PMIOPort  Port=2  Side=Right
  connections:
  Winding Conductance/RConn1 -- A/RConn1
  B/RConn1 -- Winding-Iron Conductance/RConn1 -- Iron Stack-Case Conductance/LConn1 -- Stator Iron Thermal Mass/LConn1
  Case-Ambient Insulated/LConn1 -- Iron Stack-Case Conductance/RConn1 -- Motor Case Thermal Mass/LConn1
  Winding Thermal Mass/LConn1 -- Winding Conductance/LConn1 -- Winding-Iron Conductance/LConn1

== system sm_car/Vehicle/Vehicle/Powertrain/Power/Electric L1 R1 L2 R2/Thermal/Liquid Loop1/Thermal Circuit Motor R1 ==
  Case-Ambient Insulated : fl_lib/Thermal/Thermal Elements/Perfect Insulator  T_specify=off  T_priority=None  T=0 K  T_nominal_specify=off  T_nominal_value=1  T_nominal_unit=K
  Iron Stack-Case Conductance : fl_lib/Thermal/Thermal Elements/Conductive Heat Transfer  thermal_type=foundation.enum.ConstantVariableTabulated.Constant  wall_geometry=foundation.enum.ConductionWallGeometry.Planar  area=4350 cm^2  thickness=1 cm  d_in=0.05 m  d_out=0.1 m  L=1 m  th_cond_min=10 W/(K*m)  th_cond=80.2 W/(m*K)  th_cond_TLU=[413, 401, 392, 383, 371, 357, 342] W/(K*m)  temp_TLU=[200, 273, 400, 600, 800, 1000, 1200] K  T_specify=off  T_priority=None  T=0 K  T_nominal_specify=off  T_nominal_value=1  T_nominal_unit=K  Q_specify=off  Q_priority=None  Q=0 W  Q_nominal_specify=off  Q_nominal_value=1  Q_nominal_unit=W
  Motor Case Thermal Mass : fl_lib/Thermal/Thermal Elements/Thermal Mass  mass_type=foundation.enum.constant_variable.constant  mass=5 kg  sp_heat=903 J/kg/K  mass_min=1e-6 kg  num_ports=foundation.enum.numPorts2.one  m_specify=off  m_priority=High  m=1 kg  m_nominal_specify=off  m_nominal_value=1  m_nominal_unit=kg  T_specify=off  T_priority=High  T=300 K  T_nominal_specify=off  T_nominal_value=1  T_nominal_unit=K  Q_specify=off  Q_priority=None  Q=0 W  Q_nominal_specify=off  Q_nominal_value=1  Q_nominal_unit=W
  Stator Iron Thermal Mass : fl_lib/Thermal/Thermal Elements/Thermal Mass  mass_type=foundation.enum.constant_variable.constant  mass=5 kg  sp_heat=447 J/kg/K  mass_min=1e-6 kg  num_ports=foundation.enum.numPorts2.one  m_specify=off  m_priority=High  m=1 kg  m_nominal_specify=off  m_nominal_value=1  m_nominal_unit=kg  T_specify=off  T_priority=High  T=300 K  T_nominal_specify=off  T_nominal_value=1  T_nominal_unit=K  Q_specify=off  Q_priority=None  Q=0 W  Q_nominal_specify=off  Q_nominal_value=1  Q_nominal_unit=W
  Winding Conductance : fl_lib/Thermal/Thermal Elements/Conductive Heat Transfer  thermal_type=foundation.enum.ConstantVariableTabulated.Constant  wall_geometry=foundation.enum.ConductionWallGeometry.Planar  area=250.2 cm^2  thickness=1 cm  d_in=0.05 m  d_out=0.1 m  L=1 m  th_cond_min=10 W/(K*m)  th_cond=401 W/(m*K)  th_cond_TLU=[413, 401, 392, 383, 371, 357, 342] W/(K*m)  temp_TLU=[200, 273, 400, 600, 800, 1000, 1200] K  T_specify=off  T_priority=None  T=0 K  T_nominal_specify=off  T_nominal_value=1  T_nominal_unit=K  Q_specify=off  Q_priority=None  Q=0 W  Q_nominal_specify=off  Q_nominal_value=1  Q_nominal_unit=W
  Winding Thermal Mass : fl_lib/Thermal/Thermal Elements/Thermal Mass  mass_type=foundation.enum.constant_variable.constant  mass=5 kg  sp_heat=385 J/kg/K  mass_min=1e-6 kg  num_ports=foundation.enum.numPorts2.one  m_specify=off  m_priority=High  m=1 kg  m_nominal_specify=off  m_nominal_value=1  m_nominal_unit=kg  T_specify=off  T_priority=High  T=300 K  T_nominal_specify=off  T_nominal_value=1  T_nominal_unit=K  Q_specify=off  Q_priority=None  Q=0 W  Q_nominal_specify=off  Q_nominal_value=1  Q_nominal_unit=W
  Winding-Iron Conductance : fl_lib/Thermal/Thermal Elements/Conductive Heat Transfer  thermal_type=foundation.enum.ConstantVariableTabulated.Constant  wall_geometry=foundation.enum.ConductionWallGeometry.Planar  area=250 cm^2  thickness=1 cm  d_in=0.05 m  d_out=0.1 m  L=1 m  th_cond_min=10 W/(K*m)  th_cond=360 W/(m*K)  th_cond_TLU=[413, 401, 392, 383, 371, 357, 342] W/(K*m)  temp_TLU=[200, 273, 400, 600, 800, 1000, 1200] K  T_specify=off  T_priority=None  T=0 K  T_nominal_specify=off  T_nominal_value=1  T_nominal_unit=K  Q_specify=off  Q_priority=None  Q=0 W  Q_nominal_specify=off  Q_nominal_value=1  Q_nominal_unit=W
  A : PMIOPort  Side=Left
  B : PMIOPort  Port=2  Side=Right
  connections:
  Winding Conductance/RConn1 -- A/RConn1
  B/RConn1 -- Winding-Iron Conductance/RConn1 -- Iron Stack-Case Conductance/LConn1 -- Stator Iron Thermal Mass/LConn1
  Case-Ambient Insulated/LConn1 -- Iron Stack-Case Conductance/RConn1 -- Motor Case Thermal Mass/LConn1
  Winding Thermal Mass/LConn1 -- Winding Conductance/LConn1 -- Winding-Iron Conductance/LConn1

== system sm_car/Vehicle/Vehicle/Powertrain/Power/Electric L1 R1 L2 R2/Thermal/Liquid Loop1/Thermal Circuit Motor R2 ==
  Case-Ambient Insulated : fl_lib/Thermal/Thermal Elements/Perfect Insulator  T_specify=off  T_priority=None  T=0 K  T_nominal_specify=off  T_nominal_value=1  T_nominal_unit=K
  Iron Stack-Case Conductance : fl_lib/Thermal/Thermal Elements/Conductive Heat Transfer  thermal_type=foundation.enum.ConstantVariableTabulated.Constant  wall_geometry=foundation.enum.ConductionWallGeometry.Planar  area=4350 cm^2  thickness=1 cm  d_in=0.05 m  d_out=0.1 m  L=1 m  th_cond_min=10 W/(K*m)  th_cond=80.2 W/(m*K)  th_cond_TLU=[413, 401, 392, 383, 371, 357, 342] W/(K*m)  temp_TLU=[200, 273, 400, 600, 800, 1000, 1200] K  T_specify=off  T_priority=None  T=0 K  T_nominal_specify=off  T_nominal_value=1  T_nominal_unit=K  Q_specify=off  Q_priority=None  Q=0 W  Q_nominal_specify=off  Q_nominal_value=1  Q_nominal_unit=W
  Motor Case Thermal Mass : fl_lib/Thermal/Thermal Elements/Thermal Mass  mass_type=foundation.enum.constant_variable.constant  mass=5 kg  sp_heat=903 J/kg/K  mass_min=1e-6 kg  num_ports=foundation.enum.numPorts2.one  m_specify=off  m_priority=High  m=1 kg  m_nominal_specify=off  m_nominal_value=1  m_nominal_unit=kg  T_specify=off  T_priority=High  T=300 K  T_nominal_specify=off  T_nominal_value=1  T_nominal_unit=K  Q_specify=off  Q_priority=None  Q=0 W  Q_nominal_specify=off  Q_nominal_value=1  Q_nominal_unit=W
  Stator Iron Thermal Mass : fl_lib/Thermal/Thermal Elements/Thermal Mass  mass_type=foundation.enum.constant_variable.constant  mass=5 kg  sp_heat=447 J/kg/K  mass_min=1e-6 kg  num_ports=foundation.enum.numPorts2.one  m_specify=off  m_priority=High  m=1 kg  m_nominal_specify=off  m_nominal_value=1  m_nominal_unit=kg  T_specify=off  T_priority=High  T=300 K  T_nominal_specify=off  T_nominal_value=1  T_nominal_unit=K  Q_specify=off  Q_priority=None  Q=0 W  Q_nominal_specify=off  Q_nominal_value=1  Q_nominal_unit=W
  Winding Conductance : fl_lib/Thermal/Thermal Elements/Conductive Heat Transfer  thermal_type=foundation.enum.ConstantVariableTabulated.Constant  wall_geometry=foundation.enum.ConductionWallGeometry.Planar  area=250.2 cm^2  thickness=1 cm  d_in=0.05 m  d_out=0.1 m  L=1 m  th_cond_min=10 W/(K*m)  th_cond=401 W/(m*K)  th_cond_TLU=[413, 401, 392, 383, 371, 357, 342] W/(K*m)  temp_TLU=[200, 273, 400, 600, 800, 1000, 1200] K  T_specify=off  T_priority=None  T=0 K  T_nominal_specify=off  T_nominal_value=1  T_nominal_unit=K  Q_specify=off  Q_priority=None  Q=0 W  Q_nominal_specify=off  Q_nominal_value=1  Q_nominal_unit=W
  Winding Thermal Mass : fl_lib/Thermal/Thermal Elements/Thermal Mass  mass_type=foundation.enum.constant_variable.constant  mass=5 kg  sp_heat=385 J/kg/K  mass_min=1e-6 kg  num_ports=foundation.enum.numPorts2.one  m_specify=off  m_priority=High  m=1 kg  m_nominal_specify=off  m_nominal_value=1  m_nominal_unit=kg  T_specify=off  T_priority=High  T=300 K  T_nominal_specify=off  T_nominal_value=1  T_nominal_unit=K  Q_specify=off  Q_priority=None  Q=0 W  Q_nominal_specify=off  Q_nominal_value=1  Q_nominal_unit=W
  Winding-Iron Conductance : fl_lib/Thermal/Thermal Elements/Conductive Heat Transfer  thermal_type=foundation.enum.ConstantVariableTabulated.Constant  wall_geometry=foundation.enum.ConductionWallGeometry.Planar  area=250 cm^2  thickness=1 cm  d_in=0.05 m  d_out=0.1 m  L=1 m  th_cond_min=10 W/(K*m)  th_cond=360 W/(m*K)  th_cond_TLU=[413, 401, 392, 383, 371, 357, 342] W/(K*m)  temp_TLU=[200, 273, 400, 600, 800, 1000, 1200] K  T_specify=off  T_priority=None  T=0 K  T_nominal_specify=off  T_nominal_value=1  T_nominal_unit=K  Q_specify=off  Q_priority=None  Q=0 W  Q_nominal_specify=off  Q_nominal_value=1  Q_nominal_unit=W
  A : PMIOPort  Side=Left
  B : PMIOPort  Port=2  Side=Right
  connections:
  Winding Conductance/RConn1 -- A/RConn1
  B/RConn1 -- Winding-Iron Conductance/RConn1 -- Iron Stack-Case Conductance/LConn1 -- Stator Iron Thermal Mass/LConn1
  Case-Ambient Insulated/LConn1 -- Iron Stack-Case Conductance/RConn1 -- Motor Case Thermal Mass/LConn1
  Winding Thermal Mass/LConn1 -- Winding Conductance/LConn1 -- Winding-Iron Conductance/LConn1

== system sm_car/Vehicle/Vehicle/Chassis/SuspA1/Linkage/Steer/Wheel Driven Rack 1UJoint/Driver/None ==
  q : Inport
  Body Sensor Empty : Subsystem  mask{offset_body_sensor=Vehicle.Chassis.Body.sCG.Value}
      mask prompts: offset_body_sensor "Sensor Frame Offset [x y z] (m)"
  Reference Frame : sm_lib/Frames and Transforms/Reference Frame
  Reference Frame1 : sm_lib/Frames and Transforms/Reference Frame
  Reference Frame2 : sm_lib/Frames and Transforms/Reference Frame
  Terminator : Terminator
  HandR : PMIOPort  Side=Right
  HandL : PMIOPort  Port=2  Side=Right
  Ref : PMIOPort  Port=3  Side=Left
  m : Outport  VectorParamsAs1DForOutWhenUnconnected=off
  wires:
  Body Sensor Empty/1(Body) -> m/1
  q/1 -> Terminator/1
  connections:
  Ref/RConn1 -- Reference Frame2/RConn1
  HandL/RConn1 -- Body Sensor Empty/LConn1 -- Reference Frame/RConn1
  Reference Frame1/RConn1 -- HandR/RConn1
